simulink model "test_SimulinkMdl2_qLPVMPCbeta_UIO_inside2"  (R2019b)
settings: Solver=FixedStepAuto  StartTime=0.0  StopTime=10  FixedStep=DT  RelTol=1e-3
values from neighbouring files (symbols this model uses):
  beta = [-0.13962634015954636; -0.1361356816555577; -0.13264502315156904;          -0.12915436464758037; -0.12566370614359171; -0.12217304763960307;          -0.11868238913561441; -0.11519173063162574; -0.11170107212763709;          -0.10821041362364842; -0.10471975511965977; -0.10122909661567112;          -0.097738438111682452; -0.094247779607693788; -0.09075712110370511;          -0.087266462599716474;  ...(+3598 chars)    [MdlMFile.m]
  betaLUT = 0.0 0.064193209888351435 0.11259119004615419 0.14929546421559495 0.18081611050661253 0.20926497731412011 0.23701571242082992 0.26197392072434883 0.28536133270107289 0.30770154712660031 0.32934362985133 0.35028758087526196 0.37035886727319672 0.38973202197033374 0.40858157789187255    [DD_test.sldd]    (also in exUIO_WECS.m = unique(Lin_points.Pitch))
  Cq = saveVarsMat.Cq    [MdlMFile.m]
  DT = 0.008    [LUTMFile.m]    (also in UIOLinestTr.m; exUIO_WECS.m; getFictInputMatricesOrd3M.m; initWorkspace.m)
  lambda = [0; 0.1; 0.2; 0.30000000000000004; 0.4; 0.5; 0.60000000000000009;            0.70000000000000007; 0.8; 0.9; 1; 1.1; 1.2000000000000002; 1.3;            1.4000000000000001; 1.5; 1.6; 1.7000000000000002; 1.8; 1.9000000000000001;            2; 2.1; 2.2; 2.3000000000000003; 2.4000000000000004; 2.5; 2.6;            2.7; 2.8000000000000003; 2.9000000000000004; 3; 3.1; 3.2; 3.3000000000000003;            ...(+1285 chars)    [MdlMFile.m]    (also in exLQR_hamiltonian.m = -10; koopmanKhalil.m = 1)
  lambdaCqVecLUT = 0.0 6.127061506348616E-5 0.00012254123012697232 0.00018381184519045848 0.00024508246025394464 0.00030635307531743077 0.00036762369038091696 0.00042889430544440315 0.00049016492050788928 0.00055143553557137541 0.00061270615063486154 0.00067397676569834778 0.00073524738076183392 0.00079651799582532 0.00085778861088880629 0.00091905922595229242 0.00098032984101577856 0.0010416004560792648 0.001102871    [DD_test.sldd]    (also in exUIO_WECS.m = lambdaCqVecMin : dLlambdaCqVec:lambdaCqVecMax)
  lambdaTildaMat = 14.419529569316524 14.349603210880673 12.133085869773012 9.9 8.4 7.3000000000000007 6.5 5.8000000000000007 5.4 4.9 4.6000000000000005 4.3 4.1000000000000005 3.9000000000000004 3.7 13.719392614649337 13.574357234178933 11.313379017594022 9.2598290519250313 7.9268106449449158 6.9824653636911407 6.2259000594299776 5.6530125740384722 5.1921371802911152 4.81807621242771 4.4910785109643978 4.22716815598    [DD_test.sldd]    (also in exUIO_WECS.m = lambdaCqVecMax *ones(size(lambdaCqMat)))
  Lin_points = 0.74811652133345019 0.78122947334555715 0.82586806925039735 0.88042797952230989 0.94564154658981237 1.06231329175348 1.1780905557148451 1.2402773842094346 1.254474305465946 1.2544764615597244 1.2544775037226534 1.2544778841663968 1.2544780221694662 1.2544779823335293 1.254477987181289 1.2544781738200332 1.254478189259095 1.2544780953600987 1.2544781548505395 1.2544783366942183 1.2544785605869417 1    [DD_test.sldd]    (also in LinPointsMFile.m = struct)
  multTau = 0.02    [UIOLinestTr.m]    (also in exUIO_WECS.m = 1)
  sysEst = c2d(ss(F,[T*B,K],eye(nx),[zeros(size(T*B)),H]),DT,'zoh')    [exUIO_WECS.m]
  sysEstTr : value not decoded    [DD_test.sldd]
  sysMeasDel : value not decoded    [DD_test.sldd]
  tau1 = 1/DT    [ABqL_WT_est_matlab.m]    (also in exUIO_WECS.m = 125; getFictInputMatricesOrd3M.m = 125)
  wecs = 3.0    [DD_test.sldd]    (also in MdlMFile.m = struct)
undefined symbols (not defined in the file or in its folder): Rotor_Lambda
libraries: sharedTrackingLibrary x1
settings Model: DataDictionary=DD_test.sldd  ExtModeTrigMode=oneshot  ExtModeArmWhenConnect=off  Creator=Hazim Namik  LastModifiedBy=ditt_aj
settings DataIOCC: LimitDataPoints=on  SaveFormat=Array  ReturnWorkspaceOutputs=off
settings OptimizationCC: BlockReduction=off  BooleanDataType=off  LifeSpan=inf
settings DebuggingCC: SaveWithParameterizedLinksMsg=none  UnderspecifiedInitializationDetection=Classic  MergeDetectMultiDrivingBlocksExec=none  SignalResolutionControl=TryResolveAllWithWarning  SFUnexpectedBacktrackingDiag=warning  SFNoUnconditionalDefaultTransitionDiag=warning  SFExecutionAtInitializationDiag=none  ArithmeticOperatorsInVariantConditions=warning
settings HardwareCC: ProdBitPerPointer=32  ProdBitPerSizeT=32  ProdBitPerPtrDiffT=32  ProdLargestAtomicFloat=None  ProdIntDivRoundTo=Undefined  ProdEndianess=Unspecified  ProdWordSize=32  ProdHWDeviceType=32-bit Generic  TargetUnknown=on
settings ModelReferenceCC: PropagateSignalLabelsOutOfModel=off
settings SFSimCC: SimUseLocalCustomCode=off  CustomCodeUndefinedFunction=UseInterfaceOnly
settings RTWCC: RTWUseLocalCustomCode=off
settings CodeAppCC: StateflowObjectComments=on
settings GRTTargetCC: TargetLangStandard=C89/C90 (ANSI)  GeneratePreprocessorConditionals=Disable all
settings ConfigComp: CovMetricSettings=dw  CovHtmlReporting=on  CovSaveCumulativeToWorkspaceVar=on  CovSaveSingleToWorkspaceVar=on  CovExternalEMLEnable=off

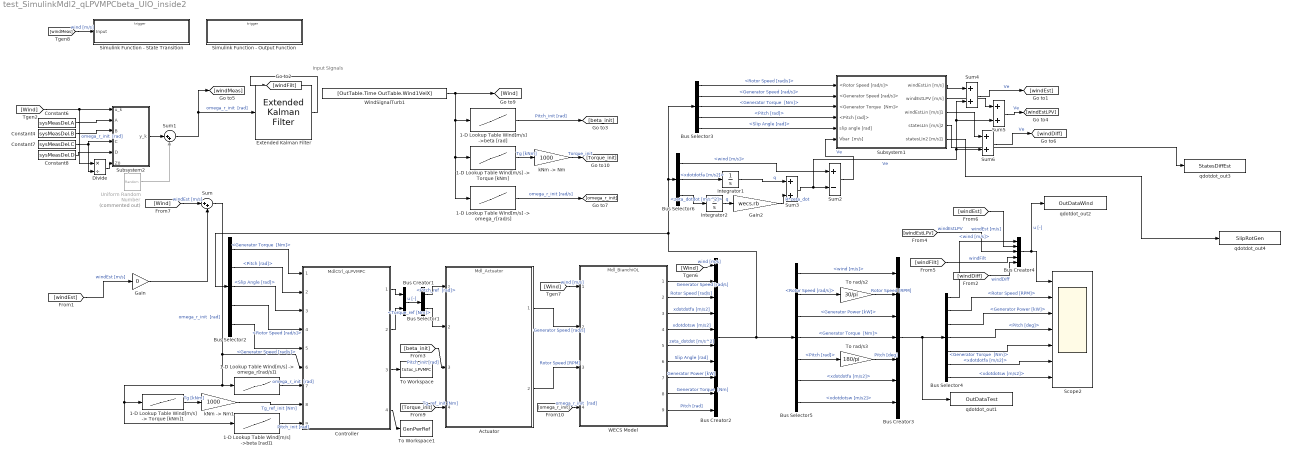
== system test_SimulinkMdl2_qLPVMPCbeta_UIO_inside2 ==
  note: Input Signals
  "1-D Lookup Table Wind[m/s] -> Torque [kNm]" : Lookup_n-D  NumberOfTableDimensions=1  BreakpointsForDimension1=Lin_points.V  BreakpointsForDimension2=Rotor_Lambda  Table=Lin_points.Torque  InternalRulePriority=Speed  RndMeth=Simplest  InputSameDT=on
  "1-D Lookup Table Wind[m/s] -> Torque [kNm]1" : Lookup_n-D  NumberOfTableDimensions=1  BreakpointsForDimension1=Lin_points.V  BreakpointsForDimension2=Rotor_Lambda  Table=Lin_points.Torque  InternalRulePriority=Speed  RndMeth=Simplest  InputSameDT=on
  "1-D Lookup Table Wind[m/s] -> omega_r[rad/s]" : Lookup_n-D  NumberOfTableDimensions=1  BreakpointsForDimension1=Lin_points.V  BreakpointsForDimension2=Rotor_Lambda  Table=Lin_points.RSpeed  InternalRulePriority=Speed  RndMeth=Simplest  InputSameDT=on
  "1-D Lookup Table Wind[m/s] -> omega_r[rad/s]1" : Lookup_n-D  NumberOfTableDimensions=1  BreakpointsForDimension1=Lin_points.V  BreakpointsForDimension2=Rotor_Lambda  Table=Lin_points.RSpeed  InternalRulePriority=Speed  RndMeth=Simplest  InputSameDT=on
  1-D Lookup Table Wind[m/s] ->beta [rad] : Lookup_n-D  NumberOfTableDimensions=1  BreakpointsForDimension1=Lin_points.V  BreakpointsForDimension2=Rotor_Lambda  Table=Lin_points.Pitch  InternalRulePriority=Speed  RndMeth=Simplest  InputSameDT=on
  1-D Lookup Table Wind[m/s] ->beta [rad]1 : Lookup_n-D  NumberOfTableDimensions=1  BreakpointsForDimension1=Lin_points.V  BreakpointsForDimension2=Rotor_Lambda  Table=Lin_points.Pitch  InternalRulePriority=Speed  RndMeth=Simplest  InputSameDT=on
  Actuator : ModelReference  ModelNameDialog=Mdl_Actuator.slx  SimulationMode=Normal  ModelReferenceVersion=1.14
  Bus Creator1 : BusCreator  Inputs=2
  Bus Creator2 : BusCreator  Inputs=10
  Bus Creator3 : BusCreator  Inputs=7
  Bus Creator4 : BusCreator  Inputs=5
  Bus Selector1 : BusSelector  OutputSignals="Pitch_ref  [rad],Torque_ref [Nm]"
  Bus Selector2 : BusSelector  OutputSignals="Generator Torque  [Nm],Pitch [rad],Slip Angle [rad],Rotor Speed [rad/s],Generator Speed [rad/s]"
  Bus Selector3 : BusSelector  OutputSignals="Rotor Speed [rad/s],Generator Speed [rad/s],Generator Torque  [Nm],Pitch [rad],Slip Angle [rad]"
  Bus Selector4 : BusSelector  OutputSignals="wind [m/s],Rotor Speed [RPM],Generator Power [kW],Pitch [deg],Generator Torque  [Nm],xdotdotfa [m/s2],xdotdotsw [m/s2]"
  Bus Selector5 : BusSelector  OutputSignals="wind [m/s],Rotor Speed [rad/s],Generator Power [kW],Generator Torque  [Nm],Pitch [rad],xdotdotfa [m/s2],xdotdotsw [m/s2]"
  Bus Selector6 : BusSelector  OutputSignals=wind [m/s],xdotdotfa [m/s2],zeta_dotdot [m/s^2]
  Constant4 : Constant  Value=sysMeasDel.B
  Constant6 : Constant  Value=sysMeasDel.A
  Constant7 : Constant  Value=sysMeasDel.C
  Constant8 : Constant  Value=sysMeasDel.D
  Controller : ModelReference  ModelNameDialog=MdlCtrl_qLPVMPC.slx  SimulationMode=Normal  ModelReferenceVersion=1.39
  Divide : Product  Inputs=*/
  Extended Kalman Filter : sharedTrackingLibrary/Extended Kalman Filter  StateTransitionFcn=stateTransitionFcn  HasStateTransitionJacobianFcn=off  StateTransitionJacobianFcn=stateTransitionJacobianFcn  HasAdditiveProcessNoise=Additive  ProcessNoise=0.1  HasTimeVaryingProcessNoise=off  HasStateTransitionFcnExtraArgument=0  InitialState=18  InitialStateCovariance=0.1  MeasurementFcn1=outputFcn  HasMeasurementJacobianFcn1=off  HasMeasurementEnablePort1=off  HasAdditiveMeasurementNoise1=Additive  MeasurementNoise1=1  HasTimeVaryingMeasurementNoise1=off  HasMeasurementFcnExtraArgument1=0  MeasurementFcn2=gpsMeasurementFcn  HasMeasurementJacobianFcn2=off  HasMeasurementEnablePort2=off  HasAdditiveMeasurementNoise2=Additive  MeasurementNoise2=[100 0; 0 100]  HasTimeVaryingMeasurementNoise2=off  HasMeasurementFcnExtraArgument2=0  MeasurementFcn3=myMeasurementFcn  HasMeasurementJacobianFcn3=off  HasMeasurementEnablePort3=off  HasAdditiveMeasurementNoise3=Additive  MeasurementNoise3=1  HasTimeVaryingMeasurementNoise3=off  HasMeasurementFcnExtraArgument3=0  MeasurementFcn4=myMeasurementFcn  HasMeasurementJacobianFcn4=off  HasMeasurementEnablePort4=off  HasAdditiveMeasurementNoise4=Additive  MeasurementNoise4=1  HasTimeVaryingMeasurementNoise4=off  HasMeasurementFcnExtraArgument4=0  MeasurementFcn5=myMeasurementFcn  HasMeasurementJacobianFcn5=off  HasMeasurementEnablePort5=off  HasAdditiveMeasurementNoise5=Additive  MeasurementNoise5=1  HasTimeVaryingMeasurementNoise5=off  HasMeasurementFcnExtraArgument5=0  EnableMultirate=off  StateTransitionFcnSampleTime=DT  MeasurementFcn1SampleTime=DT  MeasurementFcn2SampleTime=1  MeasurementFcn3SampleTime=-1  MeasurementFcn4SampleTime=-1  MeasurementFcn5SampleTime=-1  UseCurrentEstimator=off  OutputStateCovariance=off  DataType=double  SampleTime=DT  NumberOfMeasurements=1
      settings: SourceProductName=Control System Toolbox  SourceProductBaseCode=CT
  Gain : Gain  Gain=0
  Gain2 : Gain  Gain=wecs.rb
  Integrator1 : Integrator
  Integrator2 : Integrator
  Scope2 : Scope  NumInputPorts=7
      settings: Tag=Scope
  Simulink Function - Output Function : Subsystem  TreatAsAtomicUnit=on
  Simulink Function - State Transition : Subsystem  TreatAsAtomicUnit=on
  Subsystem1 : Subsystem
  Subsystem2 : Subsystem
  Sum : Sum  Inputs=|++
  Sum1 : Sum  Inputs=|++
  Sum2 : Sum  Inputs=+-
  Sum{3..6} (4 alike) : Sum
  To Workspace : ToWorkspace  VariableName=tictoc_LPVMPC  SaveFormat=Timeseries  SampleTime=-1
  To Workspace1 : ToWorkspace  VariableName=GenPwrRef  SaveFormat=Timeseries  SampleTime=-1
  To rad/s2 : Gain  Gain=30/pi
  To rad/s3 : Gain  Gain=180/pi
  Uniform Random Number : UniformRandomNumber  Commented=on
  WECS Model : ModelReference  ModelNameDialog=Mdl_BianchiOL.slx  SimulationMode=Normal  ModelReferenceVersion=1.68
  WindSignalTurb1 : FromWorkspace  VariableName=[OutTable.Time OutTable.Wind1VelX]  SampleTime=DT  OutputAfterFinalValue=Holding final value
  "kNm -> Nm" : Gain  Gain=1000
  "kNm -> Nm1" : Gain  Gain=1000
  qdotdot_out1 : ToWorkspace  VariableName=OutDataTest  SampleTime=-1
  qdotdot_out2 : ToWorkspace  VariableName=OutDataWind  SampleTime=-1
  qdotdot_out3 : ToWorkspace  VariableName=StatesDiffEst  SampleTime=-1
  qdotdot_out4 : ToWorkspace  VariableName=SlipRotGen  SampleTime=-1
  wires:
  Bus Creator1/1 -> Bus Selector1/1  "u [-]"
  Bus Selector1/2 -> Actuator/2  "<Torque_ref [Nm]>"
  WindSignalTurb1/1 -> [Wind], "1-D Lookup Table Wind[m/s] -> omega_r[rad/s]"/1, "1-D Lookup Table Wind[m/s] -> Torque [kNm]"/1, 1-D Lookup Table Wind[m/s] ->beta [rad]/1
  Bus Selector2/4 -> Controller/4  "<Rotor Speed [rad/s]>"
  Bus Selector5/3 -> Bus Creator3/3  "<Generator Power [kW]>"
  Bus Selector5/4 -> Bus Creator3/4  "<Generator Torque  [Nm]>"
  WECS Model/3 -> Bus Creator2/4  "xdotdotfa [m/s2]"
  Bus Selector4/7 -> Scope2/7  "<xdotdotsw [m/s2]>"
  "kNm -> Nm"/1 -> [Torque_init]  "Torque_init"
  To rad/s3/1 -> Bus Creator3/5  "Pitch [deg]"
  Bus Creator2/1 -> Bus Selector6/1, Bus Selector3/1, Bus Selector2/1, Bus Selector5/1
  Controller/1 -> Bus Creator1/1
  Controller/3 -> To Workspace/1
  WECS Model/2 -> Bus Creator2/3  "Rotor Speed [rad/s]"
  Actuator/2 -> WECS Model/3  "Rotor Speed [RPM]"
  Bus Selector2/3 -> Controller/3  "<Slip Angle [rad]>"
  Controller/2 -> Bus Creator1/2
  Bus Selector2/2 -> Controller/2  "<Pitch [rad]>"
  Bus Selector4/4 -> Scope2/4  "<Pitch [deg]>"
  Bus Selector4/5 -> Scope2/5  "<Generator Torque  [Nm]>"
  Bus Selector5/1 -> Bus Creator3/1  "<wind [m/s]>"
  [Wind] -> Bus Creator2/1  "wind [m/s]"
  Bus Selector5/5 -> To rad/s3/1  "<Pitch [rad]>"
  Bus Creator3/1 -> qdotdot_out1/1, Bus Selector4/1
  WECS Model/4 -> Bus Creator2/5  "xdotdotsw [m/s2]"
  [beta_init] -> Actuator/3  "Pitch_init [rad]"
  WECS Model/1 -> Bus Creator2/2  "Generator Speed [rad/s]"
  "1-D Lookup Table Wind[m/s] -> omega_r[rad/s]"/1 -> [omega_r_init]  "omega_r_init [rad/s]"
  Bus Selector1/1 -> Actuator/1  "<Pitch_ref  [rad]>"
  [Wind] -> WECS Model/1  "wind [m/s]"
  1-D Lookup Table Wind[m/s] ->beta [rad]/1 -> [beta_init]  "Pitch_init [rad]"
  Bus Selector4/6 -> Scope2/6  "<xdotdotfa [m/s2]>"
  "1-D Lookup Table Wind[m/s] -> Torque [kNm]"/1 -> "kNm -> Nm"/1  "Tg [kNm]"
  Bus Selector4/2 -> Scope2/2  "<Rotor Speed [RPM]>"
  Bus Selector5/6 -> Bus Creator3/6  "<xdotdotfa [m/s2]>"
  Bus Selector5/7 -> Bus Creator3/7  "<xdotdotsw [m/s2]>"
  To rad/s2/1 -> Bus Creator3/2  "Rotor Speed [RPM]"
  Bus Selector4/3 -> Scope2/3  "<Generator Power [kW]>"
  Bus Selector2/5 -> Controller/5  "<Generator Speed [rad/s]>"
  Bus Selector2/1 -> Controller/1  "<Generator Torque  [Nm]>"
  WECS Model/5 -> Bus Creator2/6  "zeta_dotdot [m/s^2]"
  [Torque_init] -> Actuator/4  "Tg_ref_init [Nm]"
  Actuator/1 -> WECS Model/2  "Generator Speed [rad/s]"
  [omega_r_init] -> WECS Model/4  "omega_r_init  [rad]"
  Bus Selector5/2 -> To rad/s2/1  "<Rotor Speed [rad/s]>"
  Controller/4 -> To Workspace1/1
  Bus Selector3/1 -> Subsystem1/1(<Rotor Speed [rad/s]>)  "<Rotor Speed [rad/s]>"
  Bus Selector3/2 -> Subsystem1/2(<Generator Speed [rad/s]>)  "<Generator Speed [rad/s]>"
  Bus Selector3/3 -> Subsystem1/3(<Generator Torque  [Nm]>)  "<Generator Torque  [Nm]>"
  Bus Selector3/4 -> Subsystem1/4(<Pitch [rad]>)  "<Pitch [rad]>"
  "kNm -> Nm1"/1 -> Controller/8  "Tg_ref_init [Nm]"
  "1-D Lookup Table Wind[m/s] -> omega_r[rad/s]1"/1 -> Controller/7  "omega_r_init  [rad]"
  Sum/1 -> 1-D Lookup Table Wind[m/s] ->beta [rad]1/1, "1-D Lookup Table Wind[m/s] -> Torque [kNm]1"/1, "1-D Lookup Table Wind[m/s] -> omega_r[rad/s]1"/1, Controller/6  "omega_r_init  [rad]"
  [windEst] -> Bus Creator4/2  "windEst [m/s]"
  Bus Creator4/1 -> qdotdot_out2/1, Scope2/1  "u [-]"
  "1-D Lookup Table Wind[m/s] -> Torque [kNm]1"/1 -> "kNm -> Nm1"/1  "Tg [kNm]"
  1-D Lookup Table Wind[m/s] ->beta [rad]1/1 -> Controller/9  "Pitch_init [rad]"
  Bus Selector4/1 -> Bus Creator4/1  "<wind [m/s]>"
  [windEstLPV] -> Bus Creator4/3  "windEstLPV"
  [Wind] -> Divide/1, Subsystem2/1(u_k)  "omega_r_init  [rad]"
  [windEst] -> Gain/1  "windEst [m/s]"
  Constant6/1 -> Subsystem2/2(A)
  Constant4/1 -> Subsystem2/3(B)
  Constant7/1 -> Subsystem2/4(C), Divide/2
  Constant8/1 -> Subsystem2/5(D)
  Divide/1 -> Subsystem2/6(Z0)
  [windFilt] -> Bus Creator4/4  "windFilt"
  Gain/1 -> Sum/2
  Extended Kalman Filter/1 -> [windFilt]
  [windMeas] -> Simulink Function - State Transition/1(Input)  "wind [m/s]"
  Subsystem2/1(y_k) -> Sum1/1
  Uniform Random Number/1 -> Sum1/2
  Sum1/1 -> [windMeas], Extended Kalman Filter/1  "omega_r_init  [rad]"
  Bus Selector3/5 -> Subsystem1/5(slip angle [rad])  "<Slip Angle [rad]>"
  [windDiff] -> Bus Creator4/5  "windDiff"
  [Wind] -> Sum/1  "windEst [m/s]"
  Gain2/1 -> Sum3/2  "R*zeta_dot"
  WECS Model/6 -> Bus Creator2/7  "Slip Angle [rad]"
  WECS Model/7 -> Bus Creator2/8  "Generator Power [kW]"
  WECS Model/8 -> Bus Creator2/9  "Generator Torque  [Nm]"
  WECS Model/9 -> Bus Creator2/10  "Pitch [rad]"
  Bus Selector6/2 -> Integrator1/1  "<xdotdotfa [m/s2]>"
  Integrator1/1 -> Sum3/1  "q"
  Bus Selector6/3 -> Integrator2/1  "<zeta_dotdot [m/s^2]>"
  Integrator2/1 -> Gain2/1  "q"
  Sum3/1 -> Sum6/2, Sum5/2, Sum4/2, Sum2/2  "Ve"
  Bus Selector6/1 -> Sum2/1  "<wind [m/s]>"
  Sum2/1 -> Subsystem1/6(Vbar  [m/s])  "Ve"
  Sum4/1 -> [windEst]  "Ve"
  Subsystem1/1(windEstLin [m/s]) -> Sum4/1
  Sum5/1 -> [windEstLPV]  "Ve"
  Subsystem1/2(windEstLPV [m/s]) -> Sum5/1
  Sum6/1 -> [windDiff]  "Ve"
  Subsystem1/3(windEstLin [m/s]1) -> Sum6/1
  Subsystem1/4(statesLIn [m/s]2) -> qdotdot_out3/1
  Subsystem1/5(statesLIn2 [m/s]1) -> qdotdot_out4/1

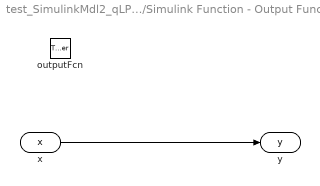
== system test_SimulinkMdl2_qLPVMPCbeta_UIO_inside2/Simulink Function - Output Function ==
  outputFcn : TriggerPort  TriggerType=function-call  IsSimulinkFunction=on  FunctionName=outputFcn  VariantControl=Variant
  x : ArgIn  DisableCoverage=on  ArgumentName=x
  y : ArgOut  DisableCoverage=on  ArgumentName=y
  wires:
  x/1 -> y/1

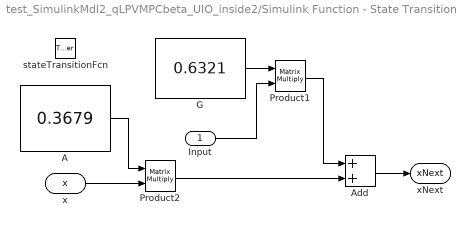
== system test_SimulinkMdl2_qLPVMPCbeta_UIO_inside2/Simulink Function - State Transition ==
  Input : Inport
  stateTransitionFcn : TriggerPort  TriggerType=function-call  IsSimulinkFunction=on  FunctionName=stateTransitionFcn  VariantControl=Variant
  A : Constant  Value=0.3679
  Add : Sum
  G : Constant  Value=0.6321
  Product1 : Product  Multiplication=Matrix(*)
  Product2 : Product  Multiplication=Matrix(*)
  x : ArgIn  DisableCoverage=on  ArgumentName=x
  xNext : ArgOut  DisableCoverage=on  ArgumentName=xNext
  wires:
  x/1 -> Product2/2
  A/1 -> Product2/1
  Product2/1 -> Add/2
  G/1 -> Product1/1
  Input/1 -> Product1/2
  Product1/1 -> Add/1
  Add/1 -> xNext/1

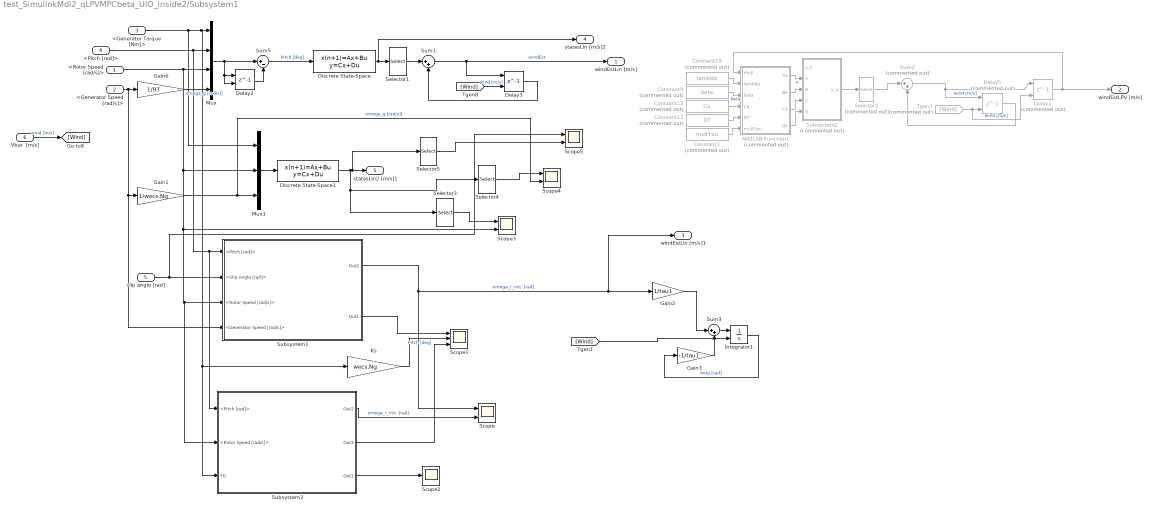
== system test_SimulinkMdl2_qLPVMPCbeta_UIO_inside2/Subsystem1 ==
  <Rotor Speed [rad/s]> : Inport
  <Generator Speed [rad/s]> : Inport  Port=2
  <Generator Torque  [Nm]> : Inport  Port=3
  <Pitch [rad]> : Inport  Port=4
  slip angle [rad] : Inport  Port=5
  Vbar  [m/s] : Inport  Port=6
  Constant1 : Constant  Commented=on  Value=multTau
  Constant10 : Constant  Commented=on  Value=lambda
  Constant11 : Constant  Commented=on  Value=DT
  Constant12 : Constant  Commented=on  Value=Cq
  Constant9 : Constant  Commented=on  Value=beta
  Delay1 : Delay  Commented=on  DelayLength=1  InitialConditionSource=Input port  InitialCondition=17.7753
      settings: InputPortMap=u0,p4
  Delay2 : Delay  DelayLength=1  InitialConditionSource=Input port  InitialCondition=0
      settings: InputPortMap=u0,p4
  Delay3 : Delay  DelayLength=1  InitialConditionSource=Input port  InitialCondition=17.7753
      settings: InputPortMap=u0,p4
  Delay5 : Delay  Commented=on  DelayLength=1  InitialConditionSource=Input port  InitialCondition=17.7753
      settings: InputPortMap=u0,p4
  Discrete State-Space : DiscreteStateSpace  A=sysEst.A  B=sysEst.B  C=sysEst.C  D=sysEst.D  SampleTime=DT
  Discrete State-Space1 : DiscreteStateSpace  A=sysEstTr.A  B=sysEstTr.B  C=sysEstTr.C  D=sysEstTr.D  InitialCondition=[0,0,1.25]  SampleTime=DT
  Gain1 : Gain  Gain=1/wecs.Ng
  Gain2 : Gain  Gain=1/tau1
  Gain3 : Gain  Gain=-1/tau1
  Gain6 : Gain  Gain=1/97
  Integrator1 : Integrator  InitialConditionSource=external
  Ks : Gain  Gain=wecs.Ng
  MATLAB Function1 : MATLAB Function  Commented=on  TreatAsAtomicUnit=on
  Mux : Mux
  Mux1 : Mux  Inputs=3
  Scope{,3..5} (4 alike) : Scope  NumInputPorts=2
  Scope1 : Scope  NumInputPorts=3
  Scope2 : Scope
  Selector1 : Selector  InputPortWidth=size(sysEst.C,1)  IndexOptions=Index vector (dialog)  Indices=size(sysEst.C,1)  OutputSizes=1
  Selector2 : Selector  Commented=on  InputPortWidth=size(sysEst.C,1)  IndexOptions=Index vector (dialog)  Indices=size(sysEst.C,1)  OutputSizes=1
  Selector3 : Selector  InputPortWidth=3  IndexOptions=Index vector (dialog)  Indices=2  OutputSizes=1
  Selector4 : Selector  InputPortWidth=3  IndexOptions=Index vector (dialog)  Indices=3  OutputSizes=1
  Selector5 : Selector  InputPortWidth=3  IndexOptions=Index vector (dialog)  Indices=1  OutputSizes=1
  Subsystem1 : Subsystem
  Subsystem2 : Subsystem  Commented=on
  Subsystem3 : Subsystem
  Sum1 : Sum  Inputs=|++
  Sum2 : Sum  Commented=on  Inputs=|++
  Sum3 : Sum  Inputs=|++
  Sum5 : Sum  Inputs=|+-
  Tgen3 : From  Commented=on  GotoTag=Wind
      settings: CloseFcn=tagdialog Close
  windEstLin [m/s] : Outport
  windEstLPV [m/s] : Outport  Port=2
  windEstLin [m/s]1 : Outport  Port=3
  statesLIn [m/s]2 : Outport  Port=4
  statesLIn2 [m/s]1 : Outport  Port=5
  wires:
  Discrete State-Space/1 -> statesLIn [m/s]2/1, Selector1/1
  Gain6/1 -> Mux/4  "omega_g [rad/s]]"
  <Generator Speed [rad/s]>/1 -> Gain1/1, Subsystem1/4(<Generator Speed [rad/s]>), Gain6/1
  Mux/1 -> Delay2/2, Delay2/1, Sum5/1
  Delay2/1 -> Sum5/2
  Selector1/1 -> Sum1/1
  Sum1/1 -> Delay3/1, windEstLin [m/s]/1  "windEst"
  Delay3/1 -> Sum1/2
  Subsystem2/1(y_k) -> Selector2/1
  MATLAB Function1/4(Dk) -> Subsystem2/5(D)
  MATLAB Function1/2(Bk) -> Subsystem2/3(B)
  Constant11/1 -> MATLAB Function1/5(DT)
  Constant10/1 -> MATLAB Function1/2(lambda)
  MATLAB Function1/3(Ck) -> Subsystem2/4(C)
  Constant9/1 -> MATLAB Function1/3(beta)  "beta"
  Constant12/1 -> MATLAB Function1/4(Cq)
  MATLAB Function1/1(Ak) -> Subsystem2/2(A)  "u"
  Vbar  [m/s]/1 -> [Wind]  "wind [m/s]"
  [Wind] -> Delay3/2  "wind [m/s]"
  Delay5/1 -> Sum2/2
  Tgen3/1 -> Delay1/2, Delay5/2  "wind [m/s]"
  Selector2/1 -> Sum2/1
  <Generator Torque  [Nm]>/1 -> Mux1/1, Ks/1, Subsystem3/3(TG), Mux/1
  <Pitch [rad]>/1 -> Subsystem1/1(<Pitch [rad]>), Subsystem3/1(<Pitch [rad]>), Mux/2
  Sum2/1 -> Delay1/1, Delay5/1  "wind [m/s]"
  Constant1/1 -> MATLAB Function1/6(multTau)
  Delay1/1 -> windEstLPV [m/s]/1, MATLAB Function1/1(rhoP)
  slip angle [rad]/1 -> Scope5/1, Subsystem1/2(<Slip Angle [rad]>)
  [Wind] -> Integrator1/2
  Sum3/1 -> Integrator1/1
  Gain3/1 -> Sum3/2
  Gain2/1 -> Sum3/1
  Integrator1/1 -> Gain3/1  "beta [rad]"
  Subsystem1/1(Out2) -> Scope/1, windEstLin [m/s]1/1, Gain2/1  "omega_r_init  [rad]"
  Sum5/1 -> Discrete State-Space/1  "Pitch [deg]"
  Subsystem3/1(Out2) -> Scope/2  "omega_r_init  [rad]"
  Subsystem1/2(Out1) -> Scope1/1
  Ks/1 -> Scope1/2  "Pitch [deg]"
  Subsystem3/3(Out1) -> Scope2/1
  Subsystem3/2(Out3) -> Scope1/3
  <Rotor Speed [rad/s]>/1 -> Mux/3, Mux1/2, Scope3/2, Subsystem3/2(<Rotor Speed [rad/s]>), Subsystem1/3(<Rotor Speed [rad/s]>)
  Mux1/1 -> Discrete State-Space1/1
  Selector3/1 -> Scope3/1
  Gain1/1 -> Scope4/2, Mux1/3  "omega_g [rad/s]]"
  Discrete State-Space1/1 -> Selector5/1, statesLIn2 [m/s]1/1, Selector4/1, Selector3/1
  Selector4/1 -> Scope4/1
  Selector5/1 -> Scope5/2

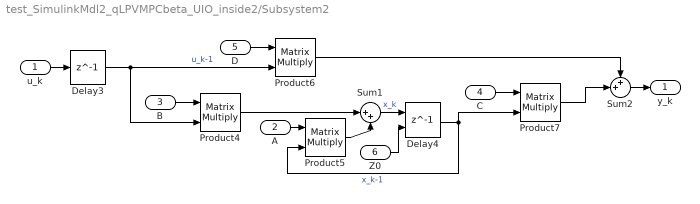
== system test_SimulinkMdl2_qLPVMPCbeta_UIO_inside2/Subsystem2 ==
  u_k : Inport
  A : Inport  Port=2
  B : Inport  Port=3
  C : Inport  Port=4
  D : Inport  Port=5
  Z0 : Inport  Port=6
  Delay3 : Delay  DelayLength=1
  Delay4 : Delay  DelayLength=1  InitialConditionSource=Input port
      settings: InputPortMap=u0,p4
  Product{4..7} (4 alike) : Product  Multiplication=Matrix(*)
  Sum1 : Sum  Inputs=|++
  Sum2 : Sum  Inputs=++|
  y_k : Outport
  wires:
  Delay4/1 -> Product7/2, Product5/2  "x_k-1"
  u_k/1 -> Delay3/1
  Product7/1 -> Sum2/2
  C/1 -> Product7/1
  Product6/1 -> Sum2/1
  Delay3/1 -> Product4/2, Product6/2  "u_k-1"
  Product5/1 -> Sum1/2
  D/1 -> Product6/1
  Product4/1 -> Sum1/1
  A/1 -> Product5/1
  Sum1/1 -> Delay4/1  "x_k"
  B/1 -> Product4/1
  Sum2/1 -> y_k/1
  Z0/1 -> Delay4/2

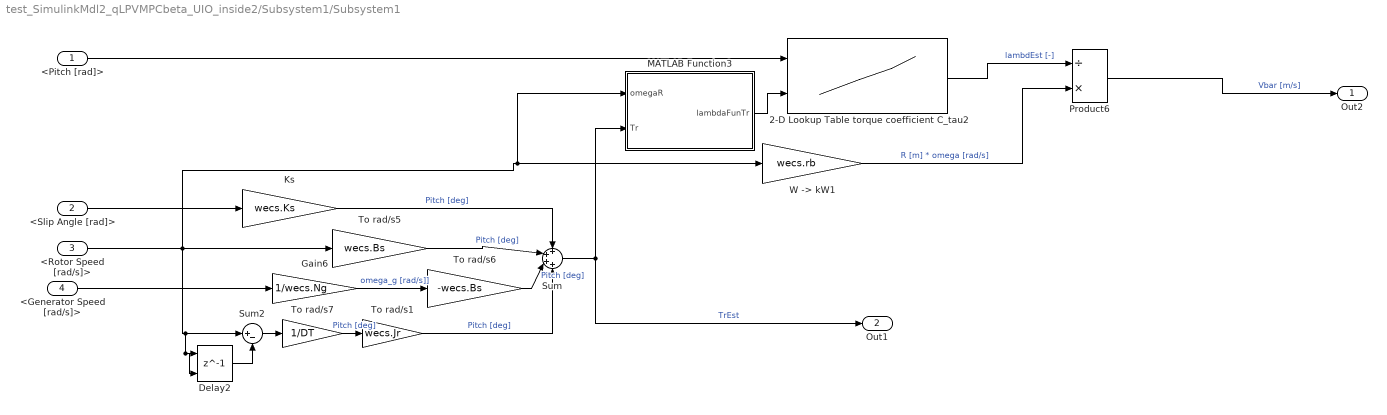
== system test_SimulinkMdl2_qLPVMPCbeta_UIO_inside2/Subsystem1/Subsystem1 ==
  <Pitch [rad]> : Inport
  <Slip Angle [rad]> : Inport  Port=2
  <Rotor Speed [rad/s]> : Inport  Port=3
  <Generator Speed [rad/s]> : Inport  Port=4
  2-D Lookup Table torque coefficient C_tau2 : Lookup_n-D  BreakpointsForDimension1=betaLUT  BreakpointsForDimension2=lambdaCqVecLUT  Table=lambdaTildaMat  InterpMethod=Cubic spline  InternalRulePriority=Speed  RndMeth=Simplest  InputSameDT=on
  Delay2 : Delay  DelayLength=1  InitialConditionSource=Input port  InitialCondition=0
      settings: InputPortMap=u0,p4
  Gain6 : Gain  Gain=1/wecs.Ng
  Ks : Gain  Gain=wecs.Ks
  MATLAB Function3 : MATLAB Function  TreatAsAtomicUnit=on
  Product6 : Product  Inputs=/*
  Sum : Sum  Inputs=4
  Sum2 : Sum  Inputs=|+-
  To rad/s1 : Gain  Gain=wecs.Jr
  To rad/s5 : Gain  Gain=wecs.Bs
  To rad/s6 : Gain  Gain=-wecs.Bs
  To rad/s7 : Gain  Gain=1/DT
  "W -> kW1" : Gain  Gain=wecs.rb
  Out2 : Outport
  Out1 : Outport  Port=2
  wires:
  2-D Lookup Table torque coefficient C_tau2/1 -> Product6/1  "lambdEst [-]"
  To rad/s1/1 -> Sum/4  "Pitch [deg]"
  Product6/1 -> Out2/1  "Vbar [m/s]"
  Sum/1 -> Out1/1, MATLAB Function3/2(Tr)  "TrEst"
  <Rotor Speed [rad/s]>/1 -> To rad/s5/1, "W -> kW1"/1, MATLAB Function3/1(omegaR), Delay2/1, Delay2/2, Sum2/1
  Sum2/1 -> To rad/s7/1
  To rad/s5/1 -> Sum/2  "Pitch [deg]"
  Delay2/1 -> Sum2/2
  MATLAB Function3/1(lambdaFunTr) -> 2-D Lookup Table torque coefficient C_tau2/2
  Gain6/1 -> To rad/s6/1  "omega_g [rad/s]]"
  To rad/s7/1 -> To rad/s1/1  "Pitch [deg]"
  To rad/s6/1 -> Sum/3  "Pitch [deg]"
  <Pitch [rad]>/1 -> 2-D Lookup Table torque coefficient C_tau2/1
  Ks/1 -> Sum/1  "Pitch [deg]"
  "W -> kW1"/1 -> Product6/2  "R [m] * omega [rad/s]"
  <Generator Speed [rad/s]>/1 -> Gain6/1
  <Slip Angle [rad]>/1 -> Ks/1

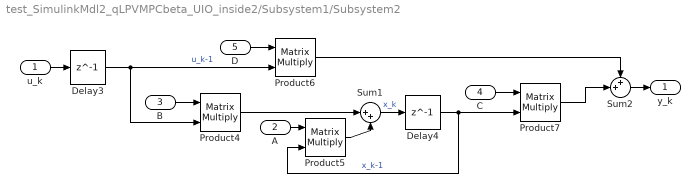
== system test_SimulinkMdl2_qLPVMPCbeta_UIO_inside2/Subsystem1/Subsystem2 ==
  u_k : Inport
  A : Inport  Port=2
  B : Inport  Port=3
  C : Inport  Port=4
  D : Inport  Port=5
  Delay3 : Delay  DelayLength=1
  Delay4 : Delay  DelayLength=1
  Product{4..7} (4 alike) : Product  Multiplication=Matrix(*)
  Sum1 : Sum  Inputs=|++
  Sum2 : Sum  Inputs=++|
  y_k : Outport
  wires:
  Delay4/1 -> Product5/2, Product7/2  "x_k-1"
  u_k/1 -> Delay3/1
  Product7/1 -> Sum2/2
  C/1 -> Product7/1
  Product6/1 -> Sum2/1
  Delay3/1 -> Product4/2, Product6/2  "u_k-1"
  Product5/1 -> Sum1/2
  D/1 -> Product6/1
  Product4/1 -> Sum1/1
  A/1 -> Product5/1
  Sum1/1 -> Delay4/1  "x_k"
  B/1 -> Product4/1
  Sum2/1 -> y_k/1

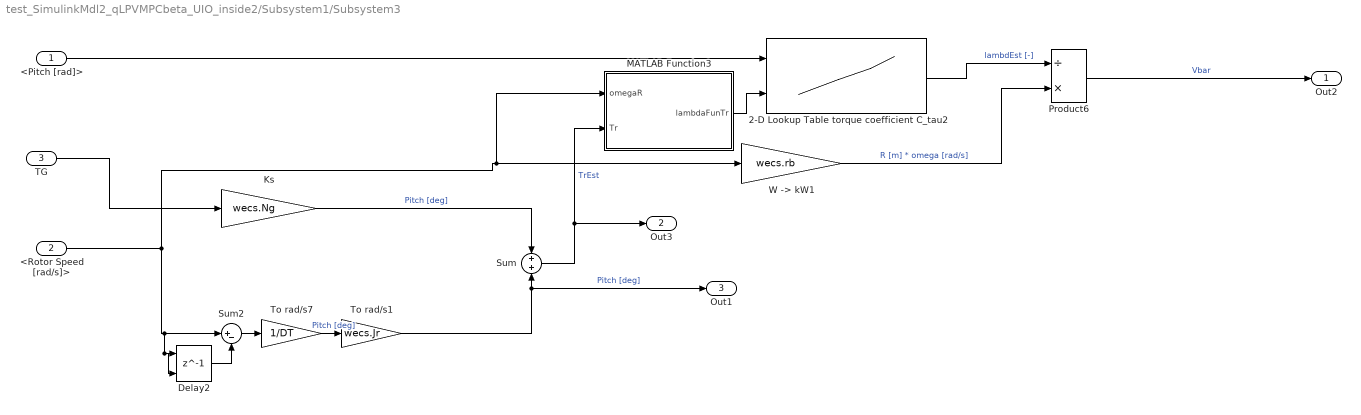
== system test_SimulinkMdl2_qLPVMPCbeta_UIO_inside2/Subsystem1/Subsystem3 ==
  <Pitch [rad]> : Inport
  <Rotor Speed [rad/s]> : Inport  Port=2
  TG : Inport  Port=3
  2-D Lookup Table torque coefficient C_tau2 : Lookup_n-D  BreakpointsForDimension1=betaLUT  BreakpointsForDimension2=lambdaCqVecLUT  Table=lambdaTildaMat  InterpMethod=Cubic spline  InternalRulePriority=Speed  RndMeth=Simplest  InputSameDT=on
  Delay2 : Delay  DelayLength=1  InitialConditionSource=Input port  InitialCondition=0
      settings: InputPortMap=u0,p4
  Ks : Gain  Gain=wecs.Ng
  MATLAB Function3 : MATLAB Function  TreatAsAtomicUnit=on
  Product6 : Product  Inputs=/*
  Sum : Sum  Inputs=2
  Sum2 : Sum  Inputs=|+-
  To rad/s1 : Gain  Gain=wecs.Jr
  To rad/s7 : Gain  Gain=1/DT
  "W -> kW1" : Gain  Gain=wecs.rb
  Out2 : Outport
  Out3 : Outport  Port=2
  Out1 : Outport  Port=3
  wires:
  2-D Lookup Table torque coefficient C_tau2/1 -> Product6/1  "lambdEst [-]"
  To rad/s1/1 -> Out1/1, Sum/2  "Pitch [deg]"
  Product6/1 -> Out2/1  "Vbar"
  Sum/1 -> Out3/1, MATLAB Function3/2(Tr)  "TrEst"
  <Rotor Speed [rad/s]>/1 -> "W -> kW1"/1, MATLAB Function3/1(omegaR), Delay2/1, Delay2/2, Sum2/1
  Sum2/1 -> To rad/s7/1
  Delay2/1 -> Sum2/2
  MATLAB Function3/1(lambdaFunTr) -> 2-D Lookup Table torque coefficient C_tau2/2
  To rad/s7/1 -> To rad/s1/1  "Pitch [deg]"
  <Pitch [rad]>/1 -> 2-D Lookup Table torque coefficient C_tau2/1
  Ks/1 -> Sum/1  "Pitch [deg]"
  "W -> kW1"/1 -> Product6/2  "R [m] * omega [rad/s]"
  TG/1 -> Ks/1

== matlab function test_SimulinkMdl2_qLPVMPCbeta_UIO_inside2/Subsystem1/Subsystem3/MATLAB Function3 ==
  data: omegaR input; Tr input; lambdaFunTr output
function lambdaFunTr = getlambdaFunTr(omegaR,Tr)

rho = 1.2250; % air density
rb = 63; % m blade radius

lambdaFunTr = 2* Tr /(rho *pi * rb^5*omegaR^2);

== matlab function test_SimulinkMdl2_qLPVMPCbeta_UIO_inside2/Subsystem1/MATLAB Function1 ==
  settings: updateMethod=DISCRETE
  data: rhoP input; lambda input; beta input; Cq input; Ak output; Bk output; DT input; Ck output; Dk output; multTau input
function [Ak,Bk,Ck,Dk]  = ABqL_WT_est(rhoP,lambda,beta,Cq,DT,multTau)
% ABqL calculates system (A) and input (B) matrix for quasiLPV
% representation for ve
%
% Inputs: * Ts: Sampling time
%         * AwithV: Scheduling parameter vector: AwithV = V
%
% Outputs: * A: System matrix A(AwithV) at current estimated air speed AwithV, discretised with Ts
%          * B: Input matrix B(AwithV) at current AwithV, discretised with Ts

% Pablo S.G. Cisneros, Herbert Werner, ICS TUHH
% modified for WECS simulation: Antje Dittmer

persistent lambdaVec pitchVec CqVec Cqdlambda Cqdbeta

if isempty(lambdaVec)
    lambdaVec =  lambda;
    pitchVec = beta;
    CqVec = Cq;
    %% Compute gradients %%[Cpdlambda,Cpdbeta] = gradient(Cp,mean(diff(Xq(1,:))),mean(diff(Yq(:,1))));
    [Cqdlambda,Cqdbeta] = gradient(CqVec,mean(diff(lambda)),mean(diff(beta))); %dcQ/dbetaDeg * dbetaDeg/dbetaRad *betaRAd
end

%% Parameters
if length(rhoP) == 1
    Vbar = rhoP; % Vbar
    LUT_V = 4:25; % LUT table rows
    
    LUT_omega = ...%[0.4815, 0.6017,0.7217,0.8413,0.9603,1.0786,1.1949, repmat(1.2671,1,15)];
        [0.7458832277625318 0.77759738173519954 0.820732502042672 ...
        0.87379091011167287 0.93538972625666472 1.0429417531956238 ...
        1.1591854391157337 1.2371015764176956 1.2554479267196832 ...
        1.2547857982936621 1.2545286368009017 1.2546177195393646 ...
        1.2545376249695805 1.2545426663335242 1.2545426663335242 ...
        1.2545426663335242 1.2545426663335242 1.2545426663335242 ...
        1.2545426663335242 1.2545426663335242 1.2545426663335242 ...
        1.2545426663335242];
    
    LUT_beta =  [0 0 0 0 0 0 0 0 0.064193209888351435 0.11259119004615419 ...
        0.14929546421559495 0.18081611050661253 0.20926497731412011 ...
        0.23701571242082992 0.26197392072434883 0.28536133270107289 ...
        0.30770154712660031 0.32934362985133 0.35028758087526196 ...
        0.37035886727319672 0.38973202197033374 0.40858157789187255 ...
        ];
    
    
    % Get omegabar and beta
    omegabar = interp1(LUT_V,LUT_omega,Vbar,'pchip');
    beta_bar = interp1(LUT_V,LUT_beta,Vbar,'pchip');
    
elseif length(rhoP) == 3
    % rho = xdotk_1([1,3,4]); % Tg not included: [Omega [1/s], beta[rad], V [m/s]];
    Vbar = rhoP(3);
    omegabar = rhoP(1); % pass OmegaR OmegaG/Ng as approximation of omegaR
    beta_bar = rhoP(2);
    
else
    error('Unexpected length of scheduling parameter rho')
end

%% Physical and model constants
rho = 1.2250;
rb = 63; % m blade radius
Ng = 97; %Gearbox ratio
Jr = (115926 + 3 * 11.776e6) *1; %kg*m^2 Inertia of the rotor (Hub inertia + 3 blades
Jg = 534.116;% * Ng^2; %kg*m^2 Inertia of the generator (HSS)
Jgr = Jg * Ng^2; % Inertia of the generator in LSS
Ks = 867637000; %Nm/rad Stiffness of the transmission
Bs = 6215000;  %Nm/rad/sec        %Damping of the transmission
tau_g = 0.01; % for pitch actuator and airspeed

%% Lambda
Lambda_bar = omegabar*rb/Vbar;
dlambdadomega= rb/Vbar;
dlambdadV = - omegabar*rb/Vbar^2;

%% Grid points
Cqb = interp2(lambdaVec,pitchVec,Cq,Lambda_bar,beta_bar);
dCqdlambdab = interp2(lambdaVec,pitchVec,Cqdlambda,Lambda_bar,beta_bar);
dCqdbetab = interp2(lambdaVec,pitchVec,Cqdbeta,Lambda_bar,beta_bar);
%% Tr=0.5*pi*rb^3*Cq*v^2
dTrdomega = 0.5*rho*pi*rb^3*(dCqdlambdab*dlambdadomega)*Vbar^2;% br = dTr/domega
dTrdbeta = 0.5*rho*pi*rb^3*dCqdbetab*Vbar^2;% Krb = dTr/dbeta
dTrdV =  2*0.5*rho*pi*rb^3*Vbar*Cqb + ...
    0.5*rho*pi*rb^3*Vbar^2*dCqdlambdab*dlambdadV;

%% Create system matrix A:
% States: [Theta_s [rad], omega_r [rad/s], omega_gr [rad/s], T_g [Nm]]
% States for model xA = [y, xdot] with y = [Tg, beta]
% x = [ThetaS, OmegaR, OmegaG, Tg, beta,]
Atemp = [[0,1,-1,0] ;
    [-Ks/Jr, (-Bs + dTrdomega)/Jr, Bs/Jr,0];
    Ks/Jgr, Bs/Jgr, -Bs/Jgr, -Ng/Jgr;
    zeros(1,3), -1/tau_g];

%% Create input matrix B
% Input orig model: V [m/s], T_g_ref [Nm], beta [rad],
% -> vel model: Vdot [m/s^2]  , T_g_refDot [Nm/s]
% for beta: Vdot [m/s^2]  T_g_refDot [Nm/s] betaDot [rad/s],
Btemp = [zeros(1,3); dTrdV/Jr, 0 dTrdbeta/Jr; zeros(1,3);  0,  1/tau_g,0];

% With Beta
AvAll = [Atemp,Btemp(:,3); zeros(1, size(Atemp,2)), -1/tau_g];
BvAll = [Btemp; zeros(1, size(Btemp,2))];
BvAll(:,3) = 0;
BvAll(end,3) = 1/tau_g;


idxS = 3;
Av = AvAll(1:idxS,1:idxS);
Bv = [BvAll(1:idxS,1),AvAll(1:idxS,idxS+1), AvAll(1:idxS,idxS+2)];


%% Check rank
Bu = Bv(:,2:3);
Bd = Bv(:,1);
nxEval = size(Av,2);

% Also create an additional state for the disturbance
tau1 =  1/DT * multTau;
A =[[Av, zeros(nxEval,1)]; [zeros(1,nxEval),-tau1]];
E = [Bd;tau1]; %xd_dot = -xd + Ed
B = [Bu; zeros(1,2)];

%% Calculate observer matrices
Ceval = [zeros(nxEval-1,1),eye(nxEval-1)]; %
nyEval = size(Ceval,1);

C = [Ceval, zeros(nyEval,1)]; %[zeros(1,nx),1]];
H = E*inv((C*E)'*(C*E))*(C*E)'; %#ok<MINV,*NOPTS> display output, inv is fast enough
nx = size(A,1);
T = eye(nx)-H*C;
A1 = T*A;

% Pole placement with Q and R
Qe = [E,B]*[E,B]'; %eye(size(A)); %B*B'; %
Re = C*C';
%K1 = lqr(A',C',Qe,Re)'; % lqr not supported in Simulink

Ham = [A', -C'* Re^(-1) * C; % Hamiltonion matrix -lambda to make it stabizable
    -Qe, -A]; 
[V,D] = eig(Ham); % Divide into stable and unstable eigenvalues
idxS = diag(D) < 0; % get stable eigenvalues
Vs = V(:,idxS);% get eigenvectors of stable eigenvalues
n11 = sum(idxS);
P = Vs(n11+1:end,:)/(Vs(1:n11,:));
K1 = real(Re^(-1) * C * P)';

% Calculate F and K
F = A1 - K1*C; %T*A -K1*C
K = K1 + F*H;
T = eye(size(H*C)) - H*C;

% Sys with no ctrl input: xdot = Ax + Ed, y = Cx  Est with no control input: zdot = Fz + Ky, xhat = z + Hy
% sysEst = ss(F,[T*B,K],eye(nx),[zeros(size(T*B)),H]); %

%% Calculate discrete forms of A,B
A2 = F*F;
A3 = F*A2;
Apre = (1.0/24.0)*DT^4*A3+(1.0/6.0)*DT^3*A2+0.5*DT^2*F+DT*eye(size(F));

%% Finish calculation of A,B
Ak = Apre*F + eye(size(F));
Bk = Apre*[T*B,K];
Ck = eye(size(F));
Dk = [zeros(size(T*B)),H];

== matlab function test_SimulinkMdl2_qLPVMPCbeta_UIO_inside2/Subsystem1/Subsystem1/MATLAB Function3 ==
  data: omegaR input; Tr input; lambdaFunTr output
function lambdaFunTr = getlambdaFunTr(omegaR,Tr)

rho = 1.2250; % air density
rb = 63; % m blade radius

lambdaFunTr = 2* Tr /(rho *pi * rb^5*omegaR^2);
